simulink model "NBMS_TTC"  (R2026b)
settings: Solver=FixedStepDiscrete  StopTime=25  FixedStep=0.1
undefined symbols (not defined in the file): BMS_MODE_E, CAL_CV_ChargeTime, CAL_DOD, CAL_SOH_Enable, Charger_Mode_Req_E
libraries: simulink x12, simulink_extras x4
settings Model: Creator=rathi  LastModifiedBy=rathi
settings OptimizationCC: DefaultParameterBehavior=Inlined  DifferentSizesBufferReuse=on  EfficientTunableParamExpr=on  EnhancedBackFolding=on  OptimizationCustomize=off  OptimizeBlockOrder=speed  PassReuseOutputArgsAs=Individual arguments  RemoveInternalMemoryZeroInit=on  RemoveRootLevelIOMemoryZeroInit=on
settings DebuggingCC: ParameterTunabilityLossMsg=error
settings SFSimCC: MATLABDynamicMemAlloc=off
settings RTWCC: Description=Embedded Coder  GenCodeOnly=on  PackageGeneratedCodeAndArtifacts=on  SystemTargetFile=ert.tlc  TemplateMakefile=ert_default_tmf
settings CodeAppCC: ForceParamTrailComments=on  IgnoreCustomStorageClasses=off  InsertBlockDesc=on  OperatorAnnotations=on  SFDataObjDesc=on  SimulinkDataObjDesc=on
settings ERTTargetCC: DynamicArrayContainerType=coder::array  GenerateSampleERTMain=on
settings ConfigComp: DVDefectChecker=on  DVDetectOutOfBounds=on  DVHarnessSource=Signal Editor  DVModelReferenceHarness=on  DVTestSuiteOptimization=Auto

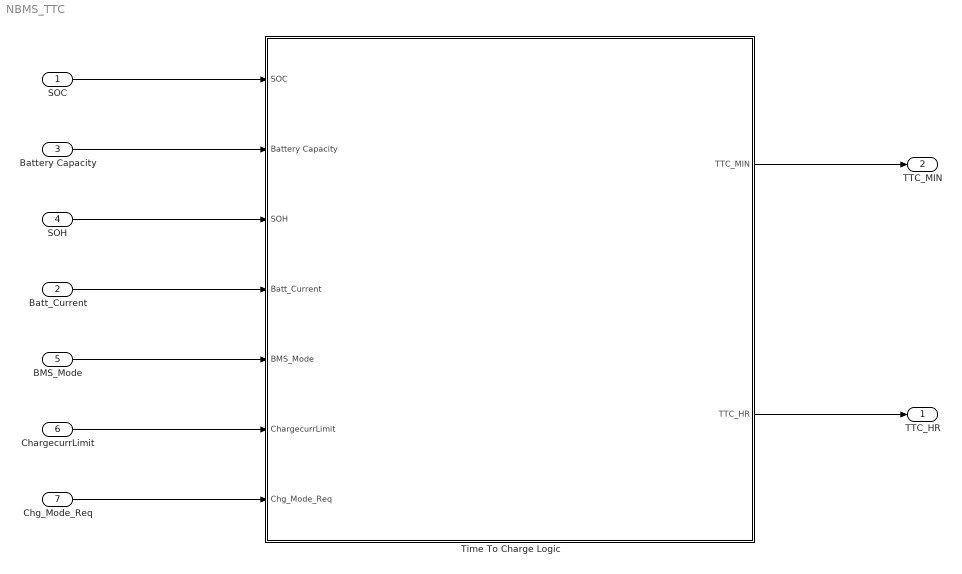
== system NBMS_TTC ==
  SOC : Inport  OutDataTypeStr=uint8
  Batt_Current : Inport  Port=2  OutDataTypeStr=fixdt(1,16,0.01,0)
  Battery Capacity : Inport  Port=3
  SOH : Inport  Port=4  OutDataTypeStr=double
  BMS_Mode : Inport  Port=5
  ChargecurrLimit : Inport  Port=6  OutDataTypeStr=double
  Chg_Mode_Req : Inport  Port=7  OutDataTypeStr=Enum: Charger_Mode_Req_E
  Time To Charge Logic : Subsystem
  TTC_HR : Outport
  TTC_MIN : Outport  Port=2
  wires:
  ChargecurrLimit/1 -> Time To Charge Logic/6(ChargecurrLimit)
  Battery Capacity/1 -> Time To Charge Logic/2(Battery Capacity)
  SOC/1 -> Time To Charge Logic/1(SOC)
  Batt_Current/1 -> Time To Charge Logic/4(Batt_Current)
  Chg_Mode_Req/1 -> Time To Charge Logic/7(Chg_Mode_Req)
  Time To Charge Logic/1(TTC_MIN) -> TTC_MIN/1
  SOH/1 -> Time To Charge Logic/3(SOH)
  Time To Charge Logic/2(TTC_HR) -> TTC_HR/1
  BMS_Mode/1 -> Time To Charge Logic/5(BMS_Mode)

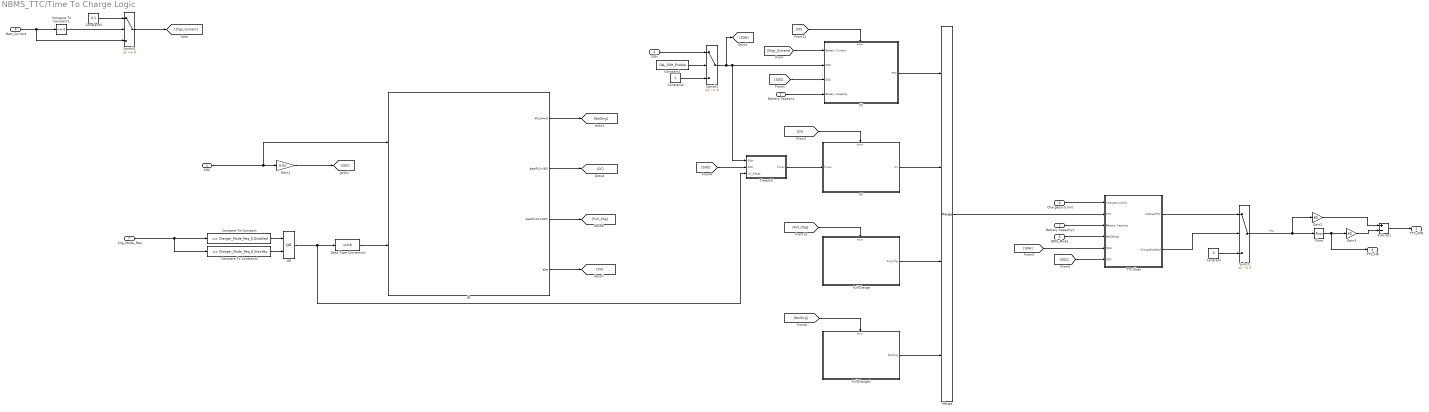
== system NBMS_TTC/Time To Charge Logic ==
  SOC : Inport  OutDataTypeStr=uint8
  Battery Capacity : Inport  Port=2
  SOH : Inport  Port=3
  Batt_Current : Inport  Port=4
  BMS_Mode : Inport  Port=5  OutDataTypeStr=Enum: BMS_MODE_E
  ChargecurrLimit : Inport  Port=6
  Chg_Mode_Req : Inport  Port=7
  Battery Capacity1 : InportShadow  Port=2
  CC : Subsystem  TreatAsAtomicUnit=on
  CV : Subsystem  TreatAsAtomicUnit=on
  Compare To Constant : simulink/Logic and Bit Operations/Compare To Constant  relop===  const=Charger_Mode_Req_E.Disabled  OutDataTypeStr=boolean
  Compare To Constant1 : simulink/Logic and Bit Operations/Compare To Constant  relop=<=  const=0  OutDataTypeStr=boolean
  Compare To Constant2 : simulink/Logic and Bit Operations/Compare To Constant  relop===  const=Charger_Mode_Req_E.Standby  OutDataTypeStr=boolean
  Constant : Constant  Value=0  OutDataTypeStr=Inherit: Inherit via back propagation
  Constant1 : Constant  Value=CAL_SOH_Enable
  Constant2 : Constant  OutDataTypeStr=Inherit: Inherit via back propagation
  Constant3 : Constant  Value=0.1  OutDataTypeStr=Inherit: Inherit via back propagation
  Data Type Conversion : DataTypeConversion  OutDataTypeStr=uint8  SaturateOnIntegerOverflow=off  RndMeth=Floor
  Floor : Rounding
  FullCharge : Subsystem  TreatAsAtomicUnit=on
  FullCharge1 : Subsystem  TreatAsAtomicUnit=on
  Gain1 : Gain  Gain=0.01
  Gain2 : Gain  Gain=60
  Gain3 : Gain  Gain=60
  If2 : If  NumInputs=2  IfExpression=u2==1  ElseIfExpressions=u1<95, u1==100
  Merge : Merge  Inputs=4
  OR : Logic  Operator=OR  AllPortsSameDT=off  OutDataTypeStr=boolean
  Subtract : Sum  Inputs=+-
  Switch : Switch  Criteria=u2 ~= 0  SaturateOnIntegerOverflow=off  InputSameDT=off
  Switch1 : Switch  Criteria=u2 ~= 0  SaturateOnIntegerOverflow=off  InputSameDT=off
  Switch2 : Switch  Criteria=u2 ~= 0  SaturateOnIntegerOverflow=off  InputSameDT=off
  TTC filter : Subsystem
  TimerCV : Subsystem
  TTC_MIN : Outport
  TTC_HR : Outport  Port=2
  wires:
  CC/1(TTC) -> Merge/1
  CV/1(CV) -> Merge/2
  Batt_Current/1 -> Switch1/3, Compare To Constant1/1
  [Chgr_Current] -> CC/1(Battery Current)
  Battery Capacity/1 -> CC/4(Battery Capacity)
  [SOC] -> CC/3(SOC)
  [SOC] -> TimerCV/2(SOC)
  [CC] -> CC/Action
  [CV] -> CV/Action
  FullCharge/1(Full_Chg) -> Merge/3
  Subtract/1 -> TTC_MIN/1
  Switch/1 -> Floor/1, Gain2/1  "TTC"
  Floor/1 -> TTC_HR/1, Gain3/1
  Gain3/1 -> Subtract/2
  Gain2/1 -> Subtract/1
  Compare To Constant1/1 -> Switch1/2
  Switch1/1 -> [Chgr_Current]
  Constant1/1 -> Switch2/2
  SOH/1 -> Switch2/1
  Constant2/1 -> Switch2/3
  Switch2/1 -> TimerCV/1(SOH), CC/2(SOH), [SOH]
  [Full_Chg] -> FullCharge/Action
  Constant3/1 -> Switch1/1
  ChargecurrLimit/1 -> TTC filter/1(ChargecurrLimit)
  Merge/1 -> TTC filter/2(TTC)
  Battery Capacity1/1 -> TTC filter/3(Battery Capacity)
  BMS_Mode/1 -> TTC filter/4(BMSMode)
  [SOH] -> TTC filter/5(SOH)
  [SOC] -> TTC filter/6(SOC)
  Chg_Mode_Req/1 -> Compare To Constant2/1, Compare To Constant/1
  If2/4 -> [CV]
  If2/3 -> [Full_Chg]
  If2/2 -> [CC]
  Compare To Constant/1 -> OR/1
  Compare To Constant2/1 -> OR/2
  OR/1 -> TimerCV/3(CV_Reset), Data Type Conversion/1
  If2/1 -> [NoChrg]
  FullCharge1/1(NoChrg) -> Merge/4
  [NoChrg] -> FullCharge1/Action
  Data Type Conversion/1 -> If2/2
  SOC/1 -> If2/1, Gain1/1
  Gain1/1 -> [SOC]
  TTC filter/2(ChargeEnabled) -> Switch/2
  TTC filter/1(FilteredTTC) -> Switch/1
  TimerCV/1(Timer) -> CV/1(Timer)
  Constant/1 -> Switch/3

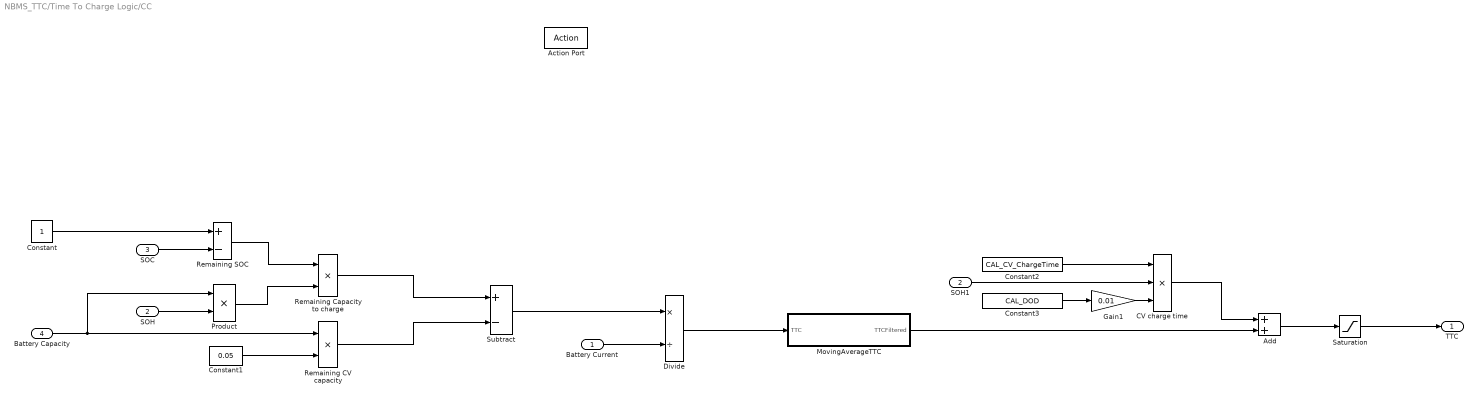
== system NBMS_TTC/Time To Charge Logic/CC ==
  Battery Current : Inport
  SOH : Inport  Port=2
  SOC : Inport  Port=3
  Battery Capacity : Inport  Port=4
  Action Port : ActionPort  ActionPortLabel=elseif(u1<95)
  Add : Sum
  CV charge time : Product  Inputs=3
  Constant : Constant
  Constant1 : Constant  Value=0.05
  Constant2 : Constant  Value=CAL_CV_ChargeTime
  Constant3 : Constant  Value=CAL_DOD
  Divide : Product  Inputs=*/
  Gain1 : Gain  Gain=0.01  OutDataTypeStr=double  RndMeth=Convergent
  MovingAverageTTC : Subsystem
  Product : Product
  Remaining CV capacity : Product
  Remaining Capacity to charge : Product
  Remaining SOC : Sum  Inputs=+-
  SOH1 : InportShadow  Port=2
  Saturation : Saturate  UpperLimit=15  LowerLimit=0
  Subtract : Sum  Inputs=+-
  TTC : Outport
  wires:
  Subtract/1 -> Divide/1
  Add/1 -> Saturation/1
  Product/1 -> Remaining Capacity to charge/2
  Remaining SOC/1 -> Remaining Capacity to charge/1
  Battery Capacity/1 -> Product/1, Remaining CV capacity/1
  SOC/1 -> Remaining SOC/2
  Constant/1 -> Remaining SOC/1
  SOH/1 -> Product/2
  Battery Current/1 -> Divide/2
  Constant1/1 -> Remaining CV capacity/2
  Saturation/1 -> TTC/1
  Constant2/1 -> CV charge time/1
  SOH1/1 -> CV charge time/2
  Constant3/1 -> Gain1/1
  Gain1/1 -> CV charge time/3
  Remaining Capacity to charge/1 -> Subtract/1
  Remaining CV capacity/1 -> Subtract/2
  Divide/1 -> MovingAverageTTC/1(TTC)
  CV charge time/1 -> Add/1
  MovingAverageTTC/1(TTCFiltered) -> Add/2

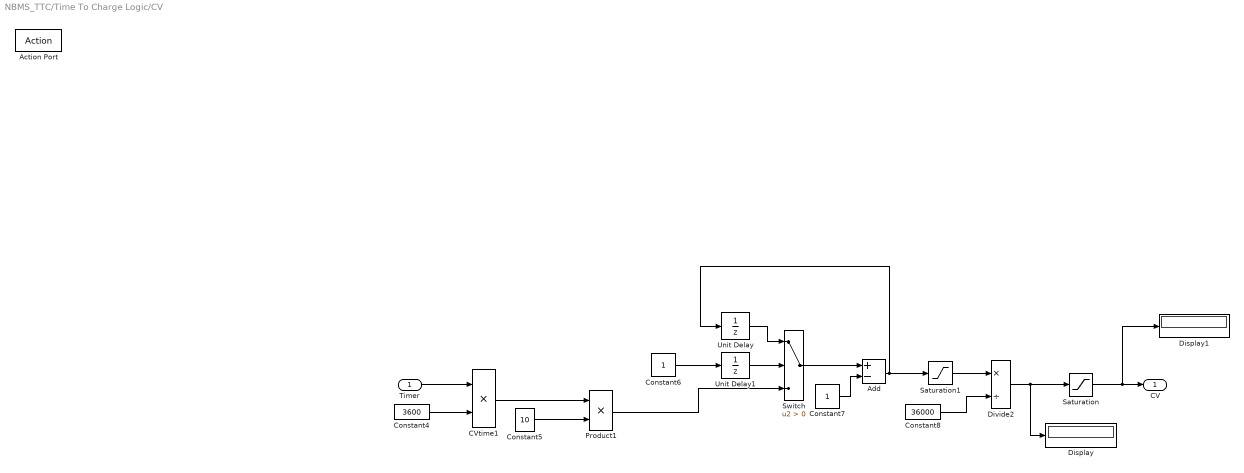
== system NBMS_TTC/Time To Charge Logic/CV ==
  Timer : Inport
  Action Port : ActionPort  ActionPortLabel=else
  Add : Sum  Inputs=+-
  CVtime1 : Product
  Constant4 : Constant  Value=3600
  Constant5 : Constant  Value=10
  Constant6 : Constant
  Constant7 : Constant
  Constant8 : Constant  Value=36000
  Display : Display
  Display1 : Display
  Divide2 : Product  Inputs=*/
  Product1 : Product
  Saturation : Saturate  UpperLimit=2  LowerLimit=0
  Saturation1 : Saturate  UpperLimit=72000  LowerLimit=600
  Switch : Switch  Criteria=u2 > Threshold  SaturateOnIntegerOverflow=off  InputSameDT=off
  Unit Delay : UnitDelay  SampleTime=-1
  Unit Delay1 : UnitDelay  SampleTime=-1
  CV : Outport
  wires:
  Saturation/1 -> Display1/1, CV/1
  Constant4/1 -> CVtime1/2
  CVtime1/1 -> Product1/1
  Constant5/1 -> Product1/2
  Unit Delay/1 -> Switch/1
  Constant6/1 -> Unit Delay1/1
  Unit Delay1/1 -> Switch/2
  Product1/1 -> Switch/3
  Switch/1 -> Add/1
  Constant7/1 -> Add/2
  Constant8/1 -> Divide2/2
  Divide2/1 -> Display/1, Saturation/1
  Add/1 -> Saturation1/1, Unit Delay/1
  Saturation1/1 -> Divide2/1
  Timer/1 -> CVtime1/1

== system NBMS_TTC/Time To Charge Logic/FullCharge ==
  Action Port : ActionPort  ActionPortLabel=elseif( u1==100)
  Constant : Constant  Value=0
  Full_Chg : Outport
  wires:
  Constant/1 -> Full_Chg/1

== system NBMS_TTC/Time To Charge Logic/FullCharge1 ==
  Action Port : ActionPort  ActionPortLabel=if(u2==1)
  Constant : Constant  Value=0
  NoChrg : Outport
  wires:
  Constant/1 -> NoChrg/1

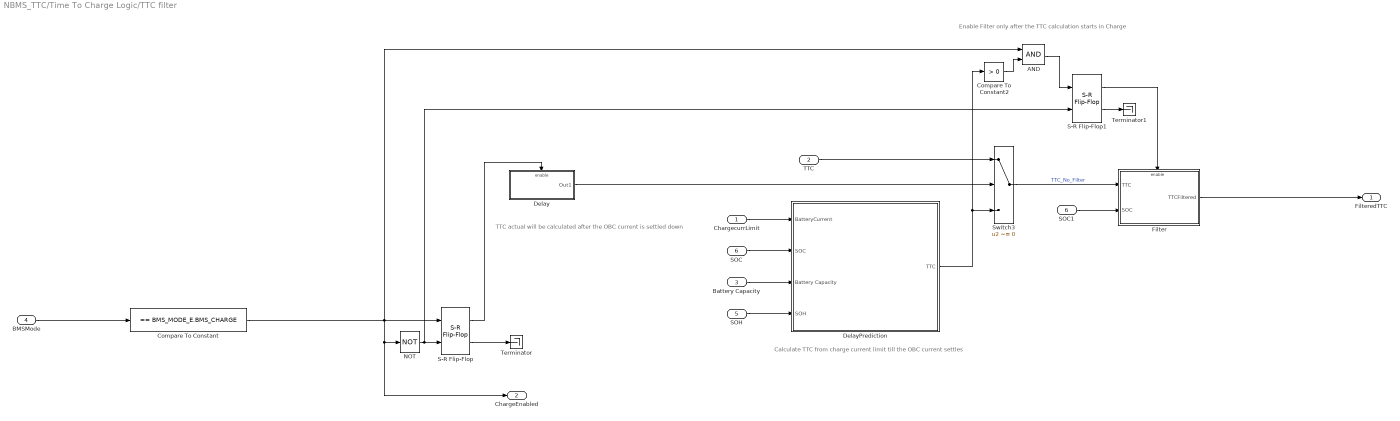
== system NBMS_TTC/Time To Charge Logic/TTC filter ==
  note: Calculate TTC from charge current limit till the OBC current settles
  note: TTC actual will be calculated after the OBC current is settled down
  note: Enable Filter only after the TTC calculation starts in Charge
  ChargecurrLimit : Inport
  TTC : Inport  Port=2
  Battery Capacity : Inport  Port=3
  BMSMode : Inport  Port=4
  SOH : Inport  Port=5
  SOC : Inport  Port=6
  AND : Logic  AllPortsSameDT=off  OutDataTypeStr=boolean
  Compare To Constant : simulink/Logic and Bit Operations/Compare To Constant  relop===  const=BMS_MODE_E.BMS_CHARGE  OutDataTypeStr=boolean
  Compare To Constant2 : simulink/Logic and Bit Operations/Compare To Constant  relop=>  const=0  OutDataTypeStr=boolean
  Delay : Subsystem  TreatAsAtomicUnit=on
  DelayPrediction : Subsystem  TreatAsAtomicUnit=on
  Filter : Subsystem  TreatAsAtomicUnit=on
  NOT : Logic  Operator=NOT  AllPortsSameDT=off  OutDataTypeStr=boolean
  S-R Flip-Flop : simulink_extras/Flip Flops/S-R Flip-Flop  initial_condition=0
  S-R Flip-Flop1 : simulink_extras/Flip Flops/S-R Flip-Flop  initial_condition=0
  SOC1 : InportShadow  Port=6
  Switch3 : Switch  Criteria=u2 ~= 0  SaturateOnIntegerOverflow=off  InputSameDT=off
  Terminator : Terminator
  Terminator1 : Terminator
  FilteredTTC : Outport
  ChargeEnabled : Outport  Port=2
  wires:
  Compare To Constant/1 -> ChargeEnabled/1, NOT/1, S-R Flip-Flop/1, AND/1
  NOT/1 -> S-R Flip-Flop1/2, S-R Flip-Flop/2
  Delay/1(Out1) -> Switch3/2
  S-R Flip-Flop/1 -> Delay/Enable
  Switch3/1 -> Filter/1(TTC)  "TTC_No_Filter"
  DelayPrediction/1(TTC) -> Compare To Constant2/1, Switch3/3
  S-R Flip-Flop/2 -> Terminator/1
  Battery Capacity/1 -> DelayPrediction/3(Battery Capacity)
  Compare To Constant2/1 -> AND/2
  ChargecurrLimit/1 -> DelayPrediction/1(BatteryCurrent)
  TTC/1 -> Switch3/1
  S-R Flip-Flop1/1 -> Filter/Enable
  AND/1 -> S-R Flip-Flop1/1
  S-R Flip-Flop1/2 -> Terminator1/1
  BMSMode/1 -> Compare To Constant/1
  Filter/1(TTCFiltered) -> FilteredTTC/1
  SOC/1 -> DelayPrediction/2(SOC)
  SOH/1 -> DelayPrediction/4(SOH)
  SOC1/1 -> Filter/2(SOC)

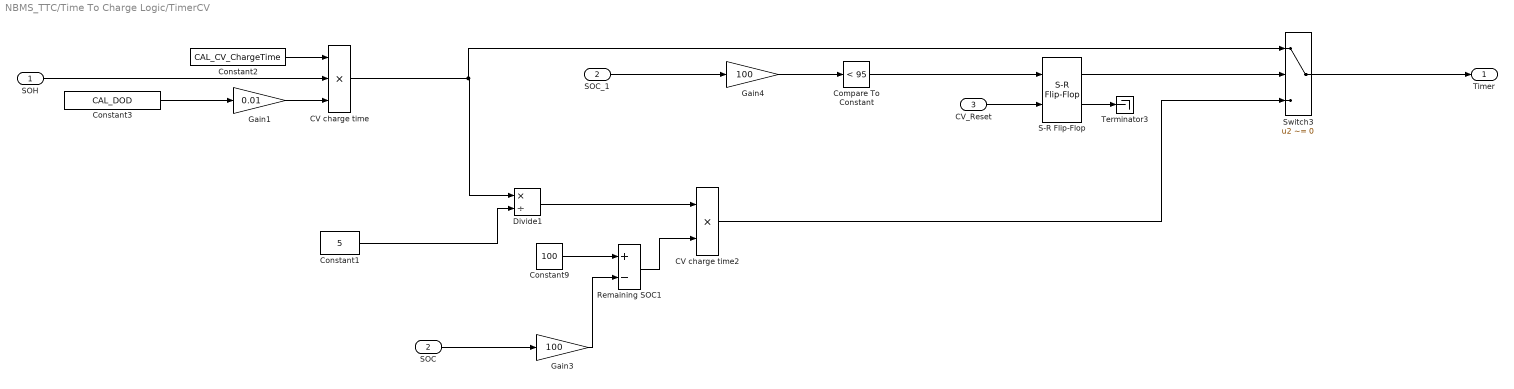
== system NBMS_TTC/Time To Charge Logic/TimerCV ==
  SOH : Inport
  SOC : Inport  Port=2
  CV_Reset : Inport  Port=3
  CV charge time : Product  Inputs=3
  CV charge time2 : Product
  Compare To Constant : simulink/Logic and Bit Operations/Compare To Constant  relop=<  const=95  OutDataTypeStr=boolean
  Constant1 : Constant  Value=5
  Constant2 : Constant  Value=CAL_CV_ChargeTime
  Constant3 : Constant  Value=CAL_DOD
  Constant9 : Constant  Value=100
  Divide1 : Product  Inputs=*/
  Gain1 : Gain  Gain=0.01  OutDataTypeStr=double  RndMeth=Convergent
  Gain3 : Gain  Gain=100  OutDataTypeStr=double  RndMeth=Convergent
  Gain4 : Gain  Gain=100  OutDataTypeStr=double  RndMeth=Convergent
  Remaining SOC1 : Sum  Inputs=+-
  S-R Flip-Flop : simulink_extras/Flip Flops/S-R Flip-Flop  initial_condition=0
  SOC_1 : InportShadow  Port=2
  Switch3 : Switch  Criteria=u2 ~= 0  SaturateOnIntegerOverflow=off  InputSameDT=off
  Terminator3 : Terminator
  Timer : Outport
  wires:
  S-R Flip-Flop/1 -> Switch3/2
  Constant2/1 -> CV charge time/1
  Compare To Constant/1 -> S-R Flip-Flop/1
  S-R Flip-Flop/2 -> Terminator3/1
  Constant3/1 -> Gain1/1
  SOH/1 -> CV charge time/2
  Remaining SOC1/1 -> CV charge time2/2
  Constant9/1 -> Remaining SOC1/1
  CV charge time/1 -> Switch3/1, Divide1/1
  Switch3/1 -> Timer/1
  Divide1/1 -> CV charge time2/1
  Gain1/1 -> CV charge time/3
  Gain4/1 -> Compare To Constant/1
  SOC/1 -> Gain3/1
  Constant1/1 -> Divide1/2
  CV charge time2/1 -> Switch3/3
  SOC_1/1 -> Gain4/1
  Gain3/1 -> Remaining SOC1/2
  CV_Reset/1 -> S-R Flip-Flop/2

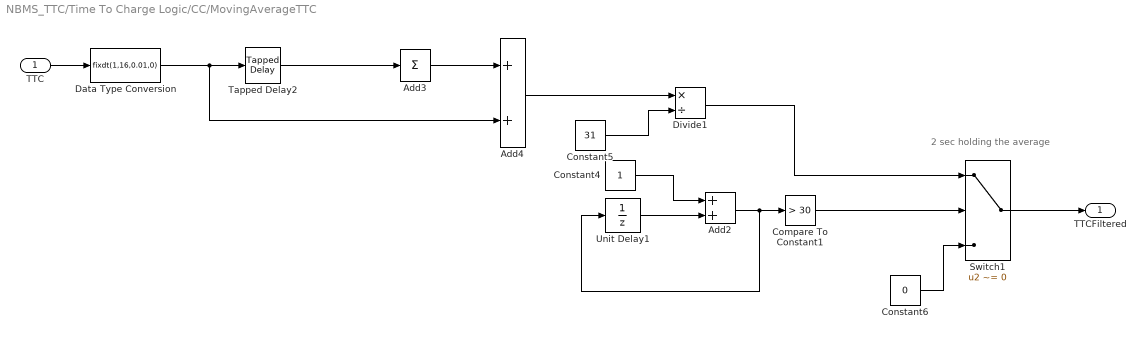
== system NBMS_TTC/Time To Charge Logic/CC/MovingAverageTTC ==
  note: 2 sec holding the average
  TTC : Inport
  Add2 : Sum  AccumDataTypeStr=uint8  SaturateOnIntegerOverflow=on
  Add3 : Sum  Inputs=+  OutDataTypeStr=fixdt(1,32,0.01,0)  AccumDataTypeStr=fixdt(1,32,0.01,0)
  Add4 : Sum  OutDataTypeStr=fixdt(1,32,0.01,0)  AccumDataTypeStr=fixdt(1,32,0.01,0)
  Compare To Constant1 : simulink/Logic and Bit Operations/Compare To Constant  relop=>  const=30  OutDataTypeStr=boolean
  Constant4 : Constant  OutDataTypeStr=uint8
  Constant5 : Constant  Value=31  OutDataTypeStr=fixdt(1,16,0.01,0)
  Constant6 : Constant  Value=0  OutDataTypeStr=fixdt(1,16,0.01,0)
  Data Type Conversion : DataTypeConversion  OutDataTypeStr=fixdt(1,16,0.01,0)  SaturateOnIntegerOverflow=off  RndMeth=Floor
  Divide1 : Product  Inputs=*/  OutDataTypeStr=fixdt(1,16,0.01,0)
  Switch1 : Switch  Criteria=u2 ~= 0  Threshold=20  SaturateOnIntegerOverflow=off  InputSameDT=off
  Tapped Delay2 : simulink/Discrete/Tapped Delay  vinit=0.0  samptime=0.1  NumDelays=30  DelayOrder=Oldest  includeCurrent=off
  Unit Delay1 : UnitDelay  SampleTime=-1
  TTCFiltered : Outport  OutputWhenDisabled=reset  InitialOutput=0
  wires:
  Divide1/1 -> Switch1/1
  Data Type Conversion/1 -> Add4/2, Tapped Delay2/1
  Unit Delay1/1 -> Add2/2
  Switch1/1 -> TTCFiltered/1
  Constant4/1 -> Add2/1
  TTC/1 -> Data Type Conversion/1
  Add4/1 -> Divide1/1
  Tapped Delay2/1 -> Add3/1
  Add3/1 -> Add4/1
  Constant5/1 -> Divide1/2
  Add2/1 -> Compare To Constant1/1, Unit Delay1/1
  Constant6/1 -> Switch1/3
  Compare To Constant1/1 -> Switch1/2

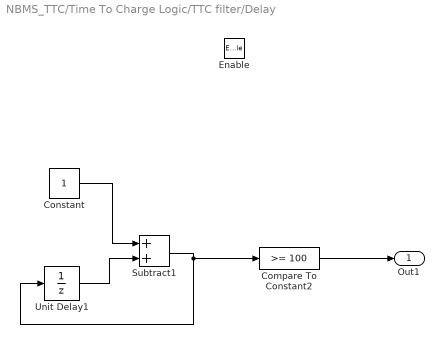
== system NBMS_TTC/Time To Charge Logic/TTC filter/Delay ==
  Enable : EnablePort  StatesWhenEnabling=reset
  Compare To Constant2 : simulink/Logic and Bit Operations/Compare To Constant  relop=>=  const=100  OutDataTypeStr=boolean
  Constant : Constant  OutDataTypeStr=uint8
  Subtract1 : Sum  OutDataTypeStr=uint8  AccumDataTypeStr=uint8  SaturateOnIntegerOverflow=on
  Unit Delay1 : UnitDelay  SampleTime=-1
  Out1 : Outport  OutputWhenDisabled=reset  InitialOutput=0
  wires:
  Subtract1/1 -> Unit Delay1/1, Compare To Constant2/1
  Unit Delay1/1 -> Subtract1/2
  Compare To Constant2/1 -> Out1/1
  Constant/1 -> Subtract1/1

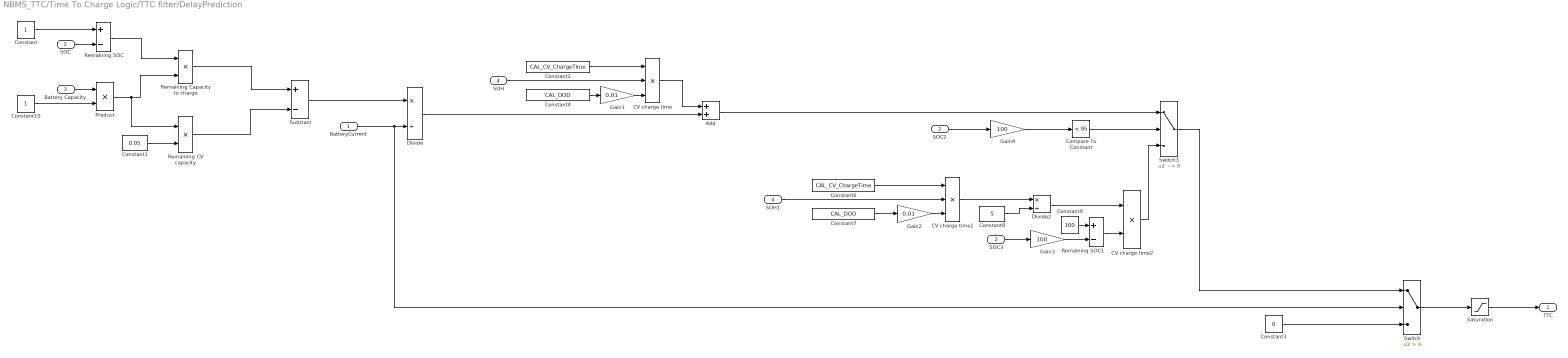
== system NBMS_TTC/Time To Charge Logic/TTC filter/DelayPrediction ==
  BatteryCurrent : Inport
  SOC : Inport  Port=2
  Battery Capacity : Inport  Port=3
  SOH : Inport  Port=4
  Add : Sum
  CV charge time : Product  Inputs=3
  CV charge time1 : Product  Inputs=3
  CV charge time2 : Product
  Compare To Constant : simulink/Logic and Bit Operations/Compare To Constant  relop=<  const=95  OutDataTypeStr=boolean
  Constant : Constant
  Constant1 : Constant  Value=0.05
  Constant10 : Constant
  Constant2 : Constant  Value=CAL_CV_ChargeTime
  Constant3 : Constant  Value=0  OutDataTypeStr=Inherit: Inherit via back propagation
  Constant4 : Constant  Value=CAL_DOD
  Constant6 : Constant  Value=CAL_CV_ChargeTime
  Constant7 : Constant  Value=CAL_DOD
  Constant8 : Constant  Value=5
  Constant9 : Constant  Value=100
  Divide : Product  Inputs=*/  SaturateOnIntegerOverflow=on
  Divide2 : Product  Inputs=*/
  Gain1 : Gain  Gain=0.01  OutDataTypeStr=double  RndMeth=Convergent
  Gain2 : Gain  Gain=0.01  OutDataTypeStr=double  RndMeth=Convergent
  Gain3 : Gain  Gain=100  OutDataTypeStr=double  RndMeth=Convergent
  Gain4 : Gain  Gain=100  OutDataTypeStr=double  RndMeth=Convergent
  Product : Product
  Remaining CV capacity : Product
  Remaining Capacity to charge : Product
  Remaining SOC : Sum  Inputs=+-
  Remaining SOC1 : Sum  Inputs=+-
  SOC2 : InportShadow  Port=2
  SOC3 : InportShadow  Port=2
  SOH1 : InportShadow  Port=4
  Saturation : Saturate  UpperLimit=15  LowerLimit=0
  Subtract : Sum  Inputs=+-
  Switch : Switch  Criteria=u2 > Threshold  SaturateOnIntegerOverflow=off  InputSameDT=off
  Switch3 : Switch  Criteria=u2 ~= 0  SaturateOnIntegerOverflow=off  InputSameDT=off
  TTC : Outport
  wires:
  Remaining Capacity to charge/1 -> Subtract/1
  Product/1 -> Remaining CV capacity/1, Remaining Capacity to charge/2
  Remaining SOC/1 -> Remaining Capacity to charge/1
  Battery Capacity/1 -> Product/1
  Divide/1 -> Add/2
  SOC/1 -> Remaining SOC/2
  Constant/1 -> Remaining SOC/1
  Remaining CV capacity/1 -> Subtract/2
  Constant1/1 -> Remaining CV capacity/2
  Saturation/1 -> TTC/1
  BatteryCurrent/1 -> Switch/2, Divide/2
  Switch/1 -> Saturation/1
  Constant3/1 -> Switch/3
  Constant2/1 -> CV charge time/1
  Constant4/1 -> Gain1/1
  SOH/1 -> CV charge time/2
  Gain1/1 -> CV charge time/3
  Subtract/1 -> Divide/1
  CV charge time/1 -> Add/1
  Add/1 -> Switch3/1
  Compare To Constant/1 -> Switch3/2
  Switch3/1 -> Switch/1
  Gain2/1 -> CV charge time1/3
  Constant7/1 -> Gain2/1
  Constant6/1 -> CV charge time1/1
  CV charge time1/1 -> Divide2/1
  Constant8/1 -> Divide2/2
  SOC2/1 -> Gain4/1
  Constant9/1 -> Remaining SOC1/1
  Remaining SOC1/1 -> CV charge time2/2
  Divide2/1 -> CV charge time2/1
  CV charge time2/1 -> Switch3/3
  SOC3/1 -> Gain3/1
  SOH1/1 -> CV charge time1/2
  Gain3/1 -> Remaining SOC1/2
  Constant10/1 -> Product/2
  Gain4/1 -> Compare To Constant/1

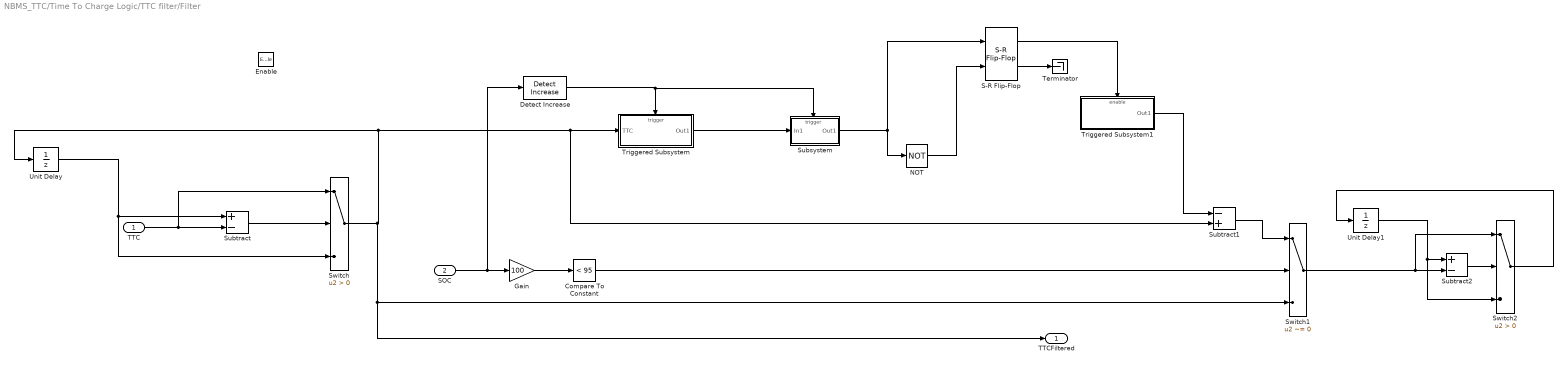
== system NBMS_TTC/Time To Charge Logic/TTC filter/Filter ==
  TTC : Inport
  SOC : Inport  Port=2
  Enable : EnablePort  StatesWhenEnabling=reset
  Compare To Constant : simulink/Logic and Bit Operations/Compare To Constant  relop=<  const=95  OutDataTypeStr=boolean
  Detect Increase : simulink/Logic and Bit Operations/Detect Increase  vinit=0.0  OutDataTypeStr=boolean
  Gain : Gain  Gain=100
  NOT : Logic  Operator=NOT  AllPortsSameDT=off  OutDataTypeStr=boolean
  S-R Flip-Flop : simulink_extras/Flip Flops/S-R Flip-Flop  initial_condition=0
  Subsystem : Subsystem
  Subtract : Sum  Inputs=+-
  Subtract1 : Sum  Inputs=-+
  Subtract2 : Sum  Inputs=+-
  Switch : Switch  Criteria=u2 > Threshold  SaturateOnIntegerOverflow=off  InputSameDT=off
  Switch1 : Switch  Criteria=u2 ~= 0  SaturateOnIntegerOverflow=off  InputSameDT=off
  Switch2 : Switch  Criteria=u2 > Threshold  SaturateOnIntegerOverflow=off  InputSameDT=off
  Terminator : Terminator
  Triggered Subsystem : Subsystem  TreatAsAtomicUnit=on
  Triggered Subsystem1 : Subsystem  TreatAsAtomicUnit=on
  Unit Delay : UnitDelay  InitialCondition=15  SampleTime=-1
  Unit Delay1 : UnitDelay  InitialCondition=15  SampleTime=-1
  TTCFiltered : Outport  OutputWhenDisabled=reset  InitialOutput=0
  wires:
  Switch/1 -> Switch1/3, TTCFiltered/1, Subtract1/2, Triggered Subsystem/1(TTC), Unit Delay/1
  TTC/1 -> Switch/1, Subtract/2
  Unit Delay/1 -> Switch/3, Subtract/1
  Subtract/1 -> Switch/2
  SOC/1 -> Detect Increase/1, Gain/1
  Gain/1 -> Compare To Constant/1
  Compare To Constant/1 -> Switch1/2
  Detect Increase/1 -> Subsystem/Trigger, Triggered Subsystem/Trigger
  S-R Flip-Flop/1 -> Triggered Subsystem1/Enable
  S-R Flip-Flop/2 -> Terminator/1
  NOT/1 -> S-R Flip-Flop/2
  Triggered Subsystem1/1(Out1) -> Subtract1/1
  Subsystem/1(Out1) -> NOT/1, S-R Flip-Flop/1
  Triggered Subsystem/1(Out1) -> Subsystem/1(In1)
  Subtract1/1 -> Switch1/1
  Switch1/1 -> Switch2/1, Subtract2/2
  Unit Delay1/1 -> Subtract2/1, Switch2/3
  Subtract2/1 -> Switch2/2
  Switch2/1 -> Unit Delay1/1

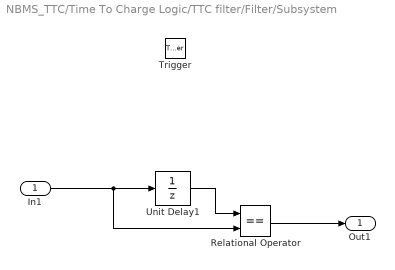
== system NBMS_TTC/Time To Charge Logic/TTC filter/Filter/Subsystem ==
  In1 : Inport
  Trigger : TriggerPort  VariantControl=(inherit)  PortDimensions=1
  Relational Operator : RelationalOperator  Operator===  OutDataTypeStr=boolean  RndMeth=Simplest  InputSameDT=off
  Unit Delay1 : UnitDelay  SampleTime=-1
  Out1 : Outport
  wires:
  Unit Delay1/1 -> Relational Operator/1
  In1/1 -> Relational Operator/2, Unit Delay1/1
  Relational Operator/1 -> Out1/1

== system NBMS_TTC/Time To Charge Logic/TTC filter/Filter/Triggered Subsystem ==
  TTC : Inport
  Trigger : TriggerPort  VariantControl=(inherit)
  Out1 : Outport
  wires:
  TTC/1 -> Out1/1

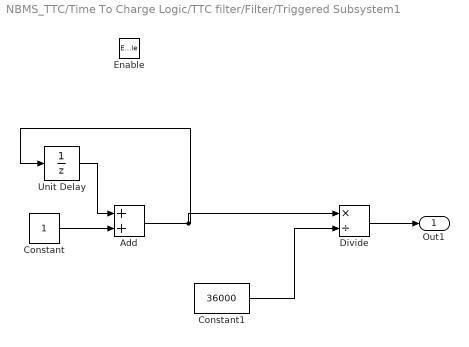
== system NBMS_TTC/Time To Charge Logic/TTC filter/Filter/Triggered Subsystem1 ==
  Enable : EnablePort
  Add : Sum
  Constant : Constant
  Constant1 : Constant  Value=36000
  Divide : Product  Inputs=*/
  Unit Delay : UnitDelay  SampleTime=-1
  Out1 : Outport
  wires:
  Constant/1 -> Add/2
  Add/1 -> Divide/1, Unit Delay/1
  Unit Delay/1 -> Add/1
  Divide/1 -> Out1/1
  Constant1/1 -> Divide/2
